simulink model "Comparaciones_consigna_vd"  (R2026b)
settings: Solver=VariableStepAuto  StopTime=3
values from neighbouring files (symbols this model uses):
  g = 9.80665    [coeficientes.m]
  T_amb = 20    [coeficientes.m]
settings Model: Creator=admin  LastModifiedBy=lamun
settings SimscapeCC: SimscapeNominalValues="[{\"value\":\"1\",\"unit\":\"A\"},{\"value\":\"1\",\"unit\":\"bar\"},{\"value\":\"1\",\"unit\":\"cm^2\"},{\"value\":\"1\",\"unit\":\"cm^3/s\"},{\"value\":\"1\",\"unit\":\"kJ/kg\"},{\"value\":\"1\",\"unit\":\"kW\"},{\"value\":\"1\",\"unit\":\"l\"},{\"value\":\"1\",\"unit\":\"N\"},{\"value\":\"1\",\"unit\":\"N*m\"},{\"value\":\"1\",\"unit\":\"V\"},{\"value\":\"0.001\",\"unit\":\"Wb\"}]"  SimscapeUseEnergyAccounting=off

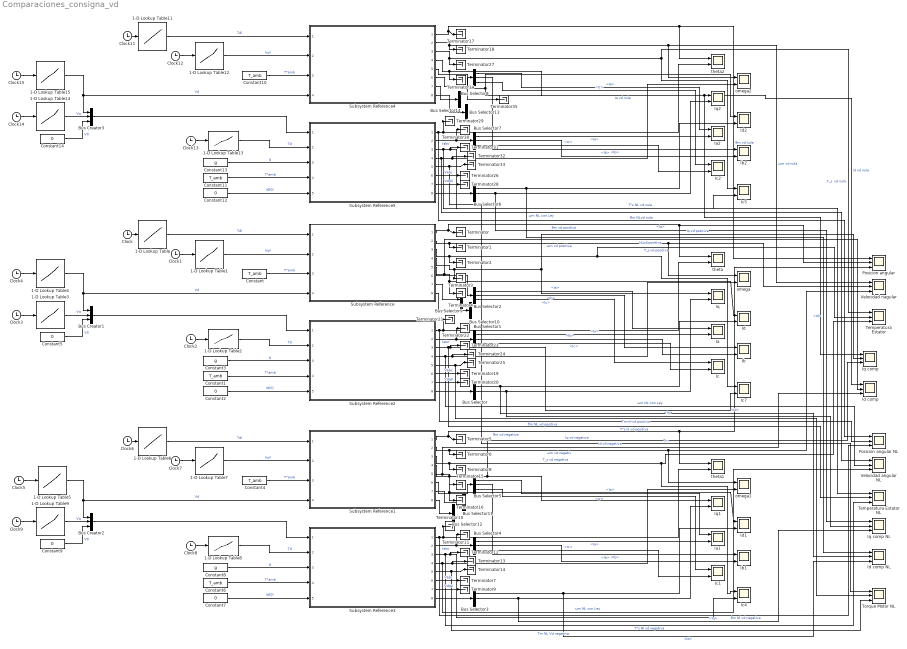
== system Comparaciones_consigna_vd ==
  " Id comp" : Scope  NumInputPorts=3
      settings: Title=Comparación de Id con distintas v*d  ActiveDisplayYMinimum=-2.0758729196219132  ActiveDisplayYMaximum=2.0758729196219132  YLabel=Corriente virtual Id  DataLoggingVariableName=ScopeData28
  " Id comp NL" : Scope  NumInputPorts=3
      settings: Title=Comparación de Id con distintas v*d MODELO NL  ActiveDisplayYMinimum=-2.0758729196219132  ActiveDisplayYMaximum=2.0758729196219132  YLabel=Corriente virtual Id  DataLoggingVariableName=ScopeData33
  " Iq comp" : Scope  NumInputPorts=3
      settings: Title=Comparación de Iq con distintas v*d  ActiveDisplayYMinimum=-14.407381995624473  ActiveDisplayYMaximum=14.636755392564851  YLabel=Corriente virtual Iq  DataLoggingVariableName=ScopeData27
  " Iq comp NL" : Scope  NumInputPorts=3
      settings: Title=Comparación de Iq con distintas v*d MODELO NL  ActiveDisplayYMinimum=-14.407381995624473  ActiveDisplayYMaximum=14.636755392564851  YLabel=Corriente virtual Iq  DataLoggingVariableName=ScopeData29
  " Temperatura Estator" : Scope  NumInputPorts=3
      settings: Title=Comparación de Temperatura estator con distintas v*d  ActiveDisplayYMinimum=-4.3883354842791764  ActiveDisplayYMaximum=39.495019358512593  YLabel=Temperatura de estator  DataLoggingVariableName=ScopeData26
  " Temperatura Estator NL" : Scope  NumInputPorts=3
      settings: Title=Comparación de Temperatura estator con distintas v*d MODELO NL  ActiveDisplayYMinimum=-4.3883354842791764  ActiveDisplayYMaximum=39.495019358512593  YLabel=Temperatura de estator  DataLoggingVariableName=ScopeData32
  " Torque Motor NL" : Scope  NumInputPorts=3
      settings: Title=Comparación de Torque Motor con distintas v*d MODELO NL  ActiveDisplayYMinimum=-1.0497695239113063  ActiveDisplayYMaximum=0.21204466447697892  YLabel=T_m [N.m]  DataLoggingVariableName=ScopeData34
  1-D Lookup Table{,2,6,8,11,13} (6 alike) : Lookup_n-D  NumberOfTableDimensions=1  BreakpointsForDimension1=[0.0, 0.1, 0.101, 0.3, 0.301, 0.5, 0.501, 0.7, 0.701, 0.9, 0.901, 1.1, 1.101, 1.3, 1.301, 1.5, 1.501, 1.7, 1.701, 1.9, 1.901, 2.0]  Table=[0.0, 0.0, 0.0, 0.0, 6.28, 6.28, -6.28, -6.28, -6.28, -6.28, 0.0, 0.0, 0.0, 0.0, 6.28, 6.28, -6.28, -6.28, 0.0, 0.0, 0.0, 0.0]  InternalRulePriority=Speed  RndMeth=Simplest
  1-D Lookup Table{1,3,7,9,12,14} (6 alike) : Lookup_n-D  NumberOfTableDimensions=1  BreakpointsForDimension1=[0.0, 0.1, 0.101, 0.3, 0.301, 0.5, 0.501, 0.7, 0.701, 0.9, 0.901, 1.1, 1.101, 1.3, 1.301, 1.5, 1.501, 1.7, 1.701, 1.9, 1.901, 2.0]  Table=[0.0, 0.0, 19.596, 19.596, 19.596, 19.596, 19.596, 19.596, 0.0, 0.0, 0.0, 0.0, -19.596, -19.596, -19.596, -19.596, -19.596, -19.596, 0.0, 0.0, 0.0, 0.0]  InternalRulePriority=Speed  RndMeth=Simplest
  1-D Lookup Table15 : Lookup_n-D  NumberOfTableDimensions=1  BreakpointsForDimension1=[0 0.5 0.5001 3]  Table=[0 0 0 0]  InternalRulePriority=Speed  RndMeth=Simplest
  1-D Lookup Table4 : Lookup_n-D  NumberOfTableDimensions=1  BreakpointsForDimension1=[0 0.5 0.5001 3]  Table=[0 0 1.9596 1.9596]  InternalRulePriority=Speed  RndMeth=Simplest
  1-D Lookup Table5 : Lookup_n-D  NumberOfTableDimensions=1  BreakpointsForDimension1=[0 0.5 0.5001 3]  Table=[0 0 -1.9596 -1.9596]  InternalRulePriority=Speed  RndMeth=Simplest
  Bus Creator1 : BusCreator  Inputs=3
  Bus Creator2 : BusCreator  Inputs=3
  Bus Creator3 : BusCreator  Inputs=3
  Bus Selector : BusSelector  OutputSignals=Id,Iq,I0
  Bus Selector{1..2,4..5,7..8} (6 alike) : BusSelector  OutputSignals=Ia,Ib,Ic
  Bus Selector10 : BusSelector  OutputSignals=Va,Vb,Vc
  Bus Selector11 : BusSelector  OutputSignals=Vd,Vq*
  Bus Selector12 : BusSelector  OutputSignals=Va,Vb,Vc
  Bus Selector13 : BusSelector  OutputSignals=Va,Vb,Vc
  Bus Selector14 : BusSelector  OutputSignals=Vd,Vq*
  Bus Selector3 : BusSelector  OutputSignals=Id,Iq,I0
  Bus Selector6 : BusSelector  OutputSignals=Id,Iq,I0
  Bus Selector9 : BusSelector  OutputSignals=Vd,Vq*
  Clock{,1..9,11..15} (15 alike) : Clock
  Constant{,1,4,6,10..11} (6 alike) : Constant  Value=T_amb
  Constant{2,5,7,9,12,14} (6 alike) : Constant  Value=0
  Constant13 : Constant  Value=g
  Constant3 : Constant  Value=g
  Constant8 : Constant  Value=g
  Ia : Scope  NumInputPorts=2
      settings: Title=Comparación Corrientes Ia  ActiveDisplayYMinimum=-15.884839257565949  ActiveDisplayYMaximum=15.842213864627638  YLabel=Corriente Ia  DataLoggingVariableName=ScopeData3
  Ia1 : Scope  NumInputPorts=2
      settings: Title=Comparación Corrientes Ia  ActiveDisplayYMinimum=-15.884839257565949  ActiveDisplayYMaximum=15.842213864627638  YLabel=Corriente Ia  DataLoggingVariableName=ScopeData8
  Ia2 : Scope  NumInputPorts=2
      settings: Title=Comparación Corrientes Ia  ActiveDisplayYMinimum=-15.884839257565949  ActiveDisplayYMaximum=15.842213864627638  YLabel=Corriente Ia  DataLoggingVariableName=ScopeData16
  Ib : Scope  NumInputPorts=2
      settings: Title=Comparación Corrientes Ib  ActiveDisplayYMinimum=-15.786152009863155  ActiveDisplayYMaximum=16.405646746971225  YLabel=Corriente Ib  DataLoggingVariableName=ScopeData4
  Ib1 : Scope  NumInputPorts=2
      settings: Title=Comparación Corrientes Ib  ActiveDisplayYMinimum=-15.786152009863155  ActiveDisplayYMaximum=16.405646746971225  YLabel=Corriente Ib  DataLoggingVariableName=ScopeData9
  Ib2 : Scope  NumInputPorts=2
      settings: Title=Comparación Corrientes Ib  ActiveDisplayYMinimum=-15.786152009863155  ActiveDisplayYMaximum=16.405646746971225  YLabel=Corriente Ib  DataLoggingVariableName=ScopeData17
  Ic{,1..2,4..5,7} (6 alike) : Scope  NumInputPorts=2
      Ic settings: Title=Comparación Corrientes Ic  ActiveDisplayYMinimum=-16.4512604006654  ActiveDisplayYMaximum=15.66373388849809  YLabel=Corriente Ic  DataLoggingVariableName=ScopeData5
      Ic1 settings: Title=Comparación Corrientes Ic  ActiveDisplayYMinimum=-16.4512604006654  ActiveDisplayYMaximum=15.66373388849809  YLabel=Corriente Ic  DataLoggingVariableName=ScopeData10
      Ic2 settings: Title=Comparación Corrientes Ic  ActiveDisplayYMinimum=-16.4512604006654  ActiveDisplayYMaximum=15.66373388849809  YLabel=Corriente Ic  DataLoggingVariableName=ScopeData18
      Ic4 settings: Title=Comparación de Temperaturas del Estator con vd* negativa  ActiveDisplayYMinimum=-4.7459661349848679  ActiveDisplayYMaximum=42.713695214863819  YLabel=Temperatura del estator  DataLoggingVariableName=ScopeData6
      Ic5 settings: Title=Comparación de Temperaturas del Estator con vd*= 0  ActiveDisplayYMinimum=-2.5502536746186673  ActiveDisplayYMaximum=22.952283071568008  YLabel=Temperatura del estator  DataLoggingVariableName=ScopeData21
      Ic7 settings: Title=Comparación de Temperaturas del Estator con vd* positiva  ActiveDisplayYMinimum=-4.4269278749266006  ActiveDisplayYMaximum=39.842350874339417  YLabel=Temperatura del estator  DataLoggingVariableName=ScopeData25
  Id : Scope  NumInputPorts=2
      settings: Title="Comparación Corrientes Viruales Id con vd*  positiva"  ActiveDisplayYMinimum=-0.25373994208722239  ActiveDisplayYMaximum=2.2836594787823734  YLabel=Corriente Virtual Id  DataLoggingVariableName=ScopeData2
  Id1 : Scope  NumInputPorts=2
      settings: Title=Comparación Corrientes Viruales Id con vd* negativa  ActiveDisplayYMinimum=-2.2835340622768117  ActiveDisplayYMaximum=0.25372600691978053  YLabel=Corriente Virtual Id  DataLoggingVariableName=ScopeData11
  Id2 : Scope  NumInputPorts=2
      settings: Title=Comparación Corrientes Viruales Id con vd* nula  ActiveDisplayYMinimum=-5  ActiveDisplayYMaximum=5  YLabel=Corriente Virtual Id  DataLoggingVariableName=ScopeData19
  Iq : Scope  NumInputPorts=2
      settings: Title=Comparación Corrientes Viruales Iq  ActiveDisplayYMinimum=-16.431377285300282  ActiveDisplayYMaximum=16.747750319569413  YLabel=Corriente Virtual Iq
  Iq1 : Scope  NumInputPorts=2
      settings: Title=Comparación Corrientes Viruales Iq  ActiveDisplayYMinimum=-16.431377285300282  ActiveDisplayYMaximum=16.747750319569413  YLabel=Corriente Virtual Iq  DataLoggingVariableName=ScopeData12
  Iq2 : Scope  NumInputPorts=2
      settings: Title=Comparación Corrientes Viruales Iq  ActiveDisplayYMinimum=-16.431377285300282  ActiveDisplayYMaximum=16.747750319569413  YLabel=Corriente Virtual Iq  DataLoggingVariableName=ScopeData20
  Posicion angular : Scope  NumInputPorts=3
      settings: Title=Comparación de posición angular con distintas v*d  ActiveDisplayYMinimum=-61.405487977979057  ActiveDisplayYMaximum=267.99815208067406  YLabel=Posición Angular [rad]  DataLoggingVariableName=ScopeData13
  Posicion angular NL : Scope  NumInputPorts=3
      settings: Title=Comparación de posición angular con distintas v*d MODELO NL  ActiveDisplayYMinimum=-61.405487977979057  ActiveDisplayYMaximum=267.99815208067406  YLabel=Posición Angular [rad]  DataLoggingVariableName=ScopeData31
  Subsystem Reference : Subsystem  ReferencedSubsystem=Modelo_LTI_Aumentado
  Subsystem Reference1 : Subsystem  ReferencedSubsystem=Modelo_LTI_Aumentado
  Subsystem Reference2 : Subsystem  ReferencedSubsystem=Modelo_LeyDeControlMinima_Complementaria
  Subsystem Reference3 : Subsystem  ReferencedSubsystem=Modelo_LeyDeControlMinima_Complementaria
  Subsystem Reference4 : Subsystem  ReferencedSubsystem=Modelo_LTI_Aumentado
  Subsystem Reference5 : Subsystem  ReferencedSubsystem=Modelo_LeyDeControlMinima_Complementaria
  Terminator{,1..35} (36 alike) : Terminator
  Velocidad angular NL : Scope  NumInputPorts=3
      settings: Title=Comparación de velocidad angular con distintas v*d MODELO NL  ActiveDisplayYMinimum=-555.23740284491123  ActiveDisplayYMaximum=527.9119503826156  YLabel=Posición Angular [rad]  DataLoggingVariableName=ScopeData30
  Velocidad nagular : Scope  NumInputPorts=3
      settings: Title=Comparación de posición angular con distintas v*d  ActiveDisplayYMinimum=-96.768856328938114  ActiveDisplayYMaximum=448.10983276139541  YLabel=Posición Angular [rad]  DataLoggingVariableName=ScopeData24
  omega : Scope  NumInputPorts=2
      settings: Title=Comparación de Velocidades Angulares  ActiveDisplayYMinimum=-564.01165677025426  ActiveDisplayYMaximum=528.88686748543148  YLabel=Velocidad Angular [rad/s]
  omega1 : Scope  NumInputPorts=2
      settings: Title=Comparación de Velocidades Angulares  ActiveDisplayYMinimum=-563.98151436747662  ActiveDisplayYMaximum=528.88351832956732  YLabel=Velocidad Angular [rad/s]  DataLoggingVariableName=ScopeData14
  omega2 : Scope  NumInputPorts=2
      settings: Title=Comparación de Velocidades Angulares  ActiveDisplayYMinimum=-562.69495517784344  ActiveDisplayYMaximum=527.40094425041116  YLabel=Velocidad Angular [rad/s]  DataLoggingVariableName=ScopeData22
  theta : Scope  NumInputPorts=2
      settings: Title=Comparación de Posiciones Angulares  ActiveDisplayYMinimum=-57.419430866655254  ActiveDisplayYMaximum=269.428234156848  YLabel=Posición Angular [rad]  DataLoggingVariableName=ScopeData7
  theta1 : Scope  NumInputPorts=2
      settings: Title=Comparación de Posiciones Angulares  ActiveDisplayYMinimum=-57.419430866655254  ActiveDisplayYMaximum=269.428234156848  YLabel=Posición Angular [rad]  DataLoggingVariableName=ScopeData15
  theta2 : Scope  NumInputPorts=2
      settings: Title=Comparación de Posiciones Angulares  ActiveDisplayYMinimum=-57.419430866655254  ActiveDisplayYMaximum=269.428234156848  YLabel=Posición Angular [rad]  DataLoggingVariableName=ScopeData23
  wires:
  Clock/1 -> 1-D Lookup Table/1
  Clock1/1 -> 1-D Lookup Table1/1
  Constant/1 -> Subsystem Reference/3  "T°amb"
  Subsystem Reference/1 -> Posicion angular/2, theta/1, Terminator/1  "θm vd positiva"
  Subsystem Reference/2 -> Terminator1/1, Velocidad nagular/2, omega/1  "ωm vd positiva"
  Subsystem Reference/3 -> " Temperatura Estator"/2, Ic7/1, Terminator2/1  "T_s vd positiva"
  Subsystem Reference/4 -> Terminator3/1, Iq/1, " Iq comp"/2  "Iq vd positiva"
  Subsystem Reference/5 -> " Id comp"/2, Terminator4/1, Id/1  "Id vd positiva"
  Constant1/1 -> Subsystem Reference2/4  "T°amb"
  Constant2/1 -> Subsystem Reference2/5  "Id(0)"
  Constant3/1 -> Subsystem Reference2/3  "g"
  1-D Lookup Table3/1 -> Bus Creator1/2  "Vq"
  Clock3/1 -> 1-D Lookup Table3/1
  Clock2/1 -> 1-D Lookup Table2/1
  1-D Lookup Table2/1 -> Subsystem Reference2/2  "Td"
  1-D Lookup Table4/1 -> Bus Creator1/1, Subsystem Reference/4  "Vd"
  Constant5/1 -> Bus Creator1/3  "V0"
  Bus Creator1/1 -> Subsystem Reference2/1
  1-D Lookup Table1/1 -> Subsystem Reference/2  "Vq*"
  1-D Lookup Table/1 -> Subsystem Reference/1  "Tdl"
  Subsystem Reference2/4 -> Velocidad angular NL/2, omega/2, Terminator24/1  "ωm NL con Ley"
  Subsystem Reference2/2 -> Terminator22/1, Bus Selector1/1  "Iabc'"
  Subsystem Reference2/5 -> " Torque Motor NL"/2, Terminator25/1  "Tm nl vd postivia"
  Subsystem Reference2/6 -> Terminator19/1  "Vabc"
  Subsystem Reference2/1 -> Posicion angular NL/2, theta/2, Terminator21/1  "θm NL vd positiva"
  Subsystem Reference2/7 -> Terminator20/1  "Vdq0"
  Subsystem Reference2/3 -> " Temperatura Estator NL"/2, Ic7/2, Terminator23/1  "T°s nl vd positiva"
  Subsystem Reference2/8 -> Bus Selector/1
  Bus Selector/2 -> " Iq comp NL"/2, Iq/2  "<Iq>"
  Bus Selector/1 -> " Id comp NL"/2, Id/2  "<Id>"
  Bus Selector1/1 -> Ia/2  "<Ia>"
  Subsystem Reference/6 -> Bus Selector2/1
  Bus Selector2/1 -> Ia/1  "<Ia>"
  Bus Selector2/2 -> Ib/1  "<Ib>"
  Bus Selector1/2 -> Ib/2  "<Ib>"
  Bus Selector2/3 -> Ic/1  "<Ic>"
  Bus Selector1/3 -> Ic/2  "<Ic>"
  Clock4/1 -> 1-D Lookup Table4/1
  1-D Lookup Table5/1 -> Bus Creator2/1, Subsystem Reference1/4  "Vd"
  Bus Selector3/2 -> " Iq comp NL"/3, Iq1/2  "<Iq>"
  Constant6/1 -> Subsystem Reference3/4  "T°amb"
  Subsystem Reference3/1 -> Posicion angular NL/3, theta1/2, Terminator10/1  "θm Nl vd negativa"
  Subsystem Reference1/4 -> Terminator15/1, " Iq comp"/3, Iq1/1  "Iq vd negativa"
  Subsystem Reference3/2 -> Terminator11/1, Bus Selector4/1  "Iabc'"
  Subsystem Reference1/6 -> Bus Selector5/1
  Clock8/1 -> 1-D Lookup Table8/1
  Clock6/1 -> 1-D Lookup Table6/1
  Subsystem Reference3/8 -> Bus Selector3/1
  Bus Selector5/2 -> Ib1/1  "<Ib>"
  Bus Selector4/1 -> Ia1/2  "<Ia>"
  Constant4/1 -> Subsystem Reference1/3  "T°amb"
  Subsystem Reference3/6 -> Terminator7/1  "Vabc"
  Subsystem Reference1/1 -> Posicion angular/3, theta1/1, Terminator5/1  "θm vd negativa"
  Subsystem Reference1/3 -> " Temperatura Estator"/3, Ic4/1, Terminator8/1  "T_s vd negativa"
  Constant9/1 -> Bus Creator2/3  "V0"
  Clock9/1 -> 1-D Lookup Table9/1
  Bus Selector3/1 -> " Id comp NL"/3, Id1/2  "<Id>"
  Subsystem Reference1/2 -> Terminator6/1, Velocidad nagular/3, omega1/1  "ωm vd negativ"
  Subsystem Reference1/5 -> " Id comp"/3, Terminator16/1, Id1/1  "Id vd negativa"
  Subsystem Reference3/7 -> Terminator9/1  "Vdq0"
  Constant7/1 -> Subsystem Reference3/5  "Id(0)"
  Subsystem Reference3/3 -> " Temperatura Estator NL"/3, Ic4/2, Terminator12/1  "T°s Nl vd negativa"
  1-D Lookup Table9/1 -> Bus Creator2/2  "Vq"
  Bus Selector5/3 -> Ic1/1  "<Ic>"
  Clock7/1 -> 1-D Lookup Table7/1
  Subsystem Reference3/5 -> " Torque Motor NL"/3, Terminator14/1  "Tm NL Vd negativa"
  1-D Lookup Table6/1 -> Subsystem Reference1/1  "Tdl"
  1-D Lookup Table8/1 -> Subsystem Reference3/2  "Td"
  Bus Selector4/3 -> Ic1/2  "<Ic>"
  Constant8/1 -> Subsystem Reference3/3  "g"
  1-D Lookup Table7/1 -> Subsystem Reference1/2  "Vq*"
  Subsystem Reference3/4 -> Velocidad angular NL/3, omega1/2, Terminator13/1  "ωm NL con Ley"
  Bus Selector5/1 -> Ia1/1  "<Ia>"
  Bus Selector4/2 -> Ib1/2  "<Ib>"
  Bus Creator2/1 -> Subsystem Reference3/1
  1-D Lookup Table15/1 -> Bus Creator3/1, Subsystem Reference4/4  "Vd"
  Bus Selector6/2 -> " Iq comp NL"/1, Iq2/2  "<Iq>"
  Constant11/1 -> Subsystem Reference5/4  "T°amb"
  Subsystem Reference5/1 -> Posicion angular NL/1, theta2/2, Terminator29/1  "θm NLvd nula"
  Subsystem Reference4/4 -> Terminator34/1, " Iq comp"/1, Iq2/1  "Iq vd nula"
  Subsystem Reference5/2 -> Terminator30/1, Bus Selector7/1  "Iabc'"
  Subsystem Reference4/6 -> Bus Selector8/1
  Clock13/1 -> 1-D Lookup Table13/1
  Clock11/1 -> 1-D Lookup Table11/1
  Subsystem Reference5/8 -> Bus Selector6/1
  Bus Selector8/2 -> Ib2/1  "<Ib>"
  Bus Selector7/1 -> Ia2/2  "<Ia>"
  Constant10/1 -> Subsystem Reference4/3  "T°amb"
  Subsystem Reference5/6 -> Terminator26/1  "Vabc"
  Subsystem Reference4/1 -> Posicion angular/1, theta2/1, Terminator17/1  "θm vd nula"
  Subsystem Reference4/3 -> Ic5/1, " Temperatura Estator"/1, Terminator27/1  "T_s  vd nula"
  Constant14/1 -> Bus Creator3/3  "V0"
  Clock14/1 -> 1-D Lookup Table14/1
  Bus Selector6/1 -> " Id comp NL"/1, Id2/2  "<Id>"
  Subsystem Reference4/2 -> Terminator18/1, Velocidad nagular/1, omega2/1  "ωm vd nula"
  Subsystem Reference4/5 -> " Id comp"/1, Id2/1, Terminator35/1  "Id vd nula"
  Subsystem Reference5/7 -> Terminator28/1  "Vdq0"
  Constant12/1 -> Subsystem Reference5/5  "Id(0)"
  Subsystem Reference5/3 -> " Temperatura Estator NL"/1, Ic5/2, Terminator31/1  "T°s NL vd nula"
  1-D Lookup Table14/1 -> Bus Creator3/2  "Vq"
  Clock15/1 -> 1-D Lookup Table15/1
  Bus Selector8/3 -> Ic2/1  "<Ic>"
  Clock12/1 -> 1-D Lookup Table12/1
  Subsystem Reference5/5 -> " Torque Motor NL"/1, Terminator33/1  "Tm"
  1-D Lookup Table11/1 -> Subsystem Reference4/1  "Tdl"
  1-D Lookup Table13/1 -> Subsystem Reference5/2  "Td"
  Bus Selector7/3 -> Ic2/2  "<Ic>"
  Constant13/1 -> Subsystem Reference5/3  "g"
  1-D Lookup Table12/1 -> Subsystem Reference4/2  "Vq*"
  Subsystem Reference5/4 -> Velocidad angular NL/1, omega2/2, Terminator32/1  "ωm NL con Ley"
  Bus Selector8/1 -> Ia2/1  "<Ia>"
  Bus Selector7/2 -> Ib2/2  "<Ib>"
  Bus Creator3/1 -> Subsystem Reference5/1
  Clock5/1 -> 1-D Lookup Table5/1
  Subsystem Reference/7 -> Bus Selector9/1
  Subsystem Reference/8 -> Bus Selector10/1
  Subsystem Reference1/7 -> Bus Selector11/1
  Subsystem Reference1/8 -> Bus Selector12/1
  Subsystem Reference4/8 -> Bus Selector13/1
  Subsystem Reference4/7 -> Bus Selector14/1
